simulink model "MATLAB_Arduino_ICM20689"  (R2021a)
settings: Solver=FixedStepAuto  StartTime=0.0  StopTime=300  RelTol=1e-3  EnableMultiTasking=on
undefined symbols (not defined in the file or in its folder): DiscIntNeverNeededParam
libraries: arduinolib x10
settings Model: SILPILModeSetting=veronly  ExtModeTrigDuration=2  Creator=mpnoy  LastModifiedBy=mpnoy
settings OptimizationCC: EnhancedBackFolding=on  PassReuseOutputArgsAs=Individual arguments  ZeroExternalMemoryAtStartup=off  ZeroInternalMemoryAtStartup=off  MaxStackSize=64  OptimizeBlockOrder=speed  DifferentSizesBufferReuse=on  OptimizationCustomize=off  EfficientTunableParamExpr=on
settings DebuggingCC: ParameterTunabilityLossMsg=error
settings HardwareCC: ProdBitPerInt=16  ProdBitPerPointer=16  ProdBitPerSizeT=16  ProdBitPerPtrDiffT=16  ProdLargestAtomicFloat=None  ProdWordSize=8  ProdHWDeviceType=Atmel->AVR
settings SFSimCC: MATLABDynamicMemAlloc=off
settings RTWCC: SystemTargetFile=ert.tlc  HardwareBoard=Arduino Uno  TemplateMakefile=ert_default_tmf  Toolchain=Arduino AVR  BuildConfiguration=Faster Runs
settings CodeAppCC: ForceParamTrailComments=on  IgnoreCustomStorageClasses=off  OperatorAnnotations=on  SimulinkDataObjDesc=on  SFDataObjDesc=on  InsertBlockDesc=on
settings ERTTargetCC: SupportContinuousTime=on  SupportVariableSizeSignals=on  ExtModeStaticAllocSize=250

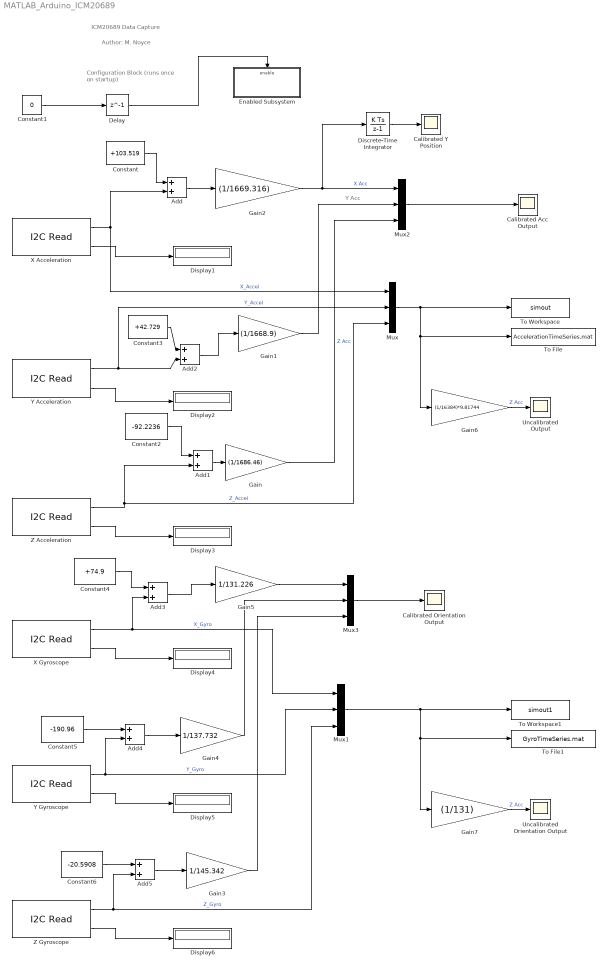
== system MATLAB_Arduino_ICM20689 ==
  note: Y Acc
  note: Author: M. Noyce
  note: ICM20689 Data Capture
  note: Configuration Block
      | (runs once on startup)
  Add{,1..5} (6 alike) : Sum
  "Calibrated Acc Output " : Scope
  Calibrated Orientation Output : Scope
  Calibrated Y Position : Scope
  Constant : Constant  Value=+103.519
  Constant1 : Constant  Value=0
  Constant2 : Constant  Value=-92.2236
  Constant3 : Constant  Value=+42.729
  Constant4 : Constant  Value=+74.9
  Constant5 : Constant  Value=-190.96
  Constant6 : Constant  Value=-20.5908
  Delay : Delay  DelayLength=1  InitialCondition=1
  Discrete-Time Integrator : DiscreteIntegrator  SampleTime=-1  ICPrevOutput=DiscIntNeverNeededParam  ICPrevScaledInput=DiscIntNeverNeededParam
  Display{1..6} (6 alike) : Display
  Enabled Subsystem : Subsystem  TreatAsAtomicUnit=on
  Gain : Gain  Gain=(1/1686.46)
  Gain1 : Gain  Gain=(1/1668.9)
  Gain2 : Gain  Gain=(1/1669.316)
  Gain3 : Gain  Gain=1/145.342
  Gain4 : Gain  Gain=1/137.732
  Gain5 : Gain  Gain=1/131.226
  Gain6 : Gain  Gain=(1/16384)*9.81744
  Gain7 : Gain  Gain=(1/131)
  Mux{,1..3} (4 alike) : Mux  Inputs=3
  To File : ToFile  Filename=AccelerationTimeSeries.mat  MatrixName=Acceleration  SaveFormat=Timeseries
  To File1 : ToFile  Filename=GyroTimeSeries.mat  MatrixName=Orientation  SaveFormat=Timeseries
  To Workspace : ToWorkspace  VariableName=simout  SaveFormat=Timeseries  SampleTime=-1
  To Workspace1 : ToWorkspace  VariableName=simout1  SaveFormat=Timeseries  SampleTime=-1
  "Uncalibrated Orientation Output " : Scope
  "Uncalibrated Output " : Scope
  "X Acceleration " : arduinolib/I2C Read  I2CModule=0  Mode=Master  SlaveAddress=104  SlaveByteOrder=BigEndian  Direction=Receiver  RegisterAddressMode=on  RegisterAddress=uint8(hex2dec('3B'))  SlaveDataType=int16  DataLength=1  NoAck=off  RepeatedStart=off  OutputStatus=on  blockPlatform=ARDUINO  SampleTime=0.01
      settings: SourceProductBaseCode=ARDUINO
  X Gyroscope : arduinolib/I2C Read  I2CModule=0  Mode=Master  SlaveAddress=104  SlaveByteOrder=BigEndian  Direction=Receiver  RegisterAddressMode=on  RegisterAddress=uint8(hex2dec('43'))  SlaveDataType=int16  DataLength=1  NoAck=off  RepeatedStart=off  OutputStatus=on  blockPlatform=ARDUINO  SampleTime=0.01
      settings: SourceProductBaseCode=ARDUINO
  Y Acceleration : arduinolib/I2C Read  I2CModule=0  Mode=Master  SlaveAddress=104  SlaveByteOrder=BigEndian  Direction=Receiver  RegisterAddressMode=on  RegisterAddress=uint8(hex2dec('3D'))  SlaveDataType=int16  DataLength=1  NoAck=off  RepeatedStart=off  OutputStatus=on  blockPlatform=ARDUINO  SampleTime=0.01
      settings: SourceProductBaseCode=ARDUINO
  Y Gyroscope : arduinolib/I2C Read  I2CModule=0  Mode=Master  SlaveAddress=104  SlaveByteOrder=BigEndian  Direction=Receiver  RegisterAddressMode=on  RegisterAddress=uint8(hex2dec('45'))  SlaveDataType=int16  DataLength=1  NoAck=off  RepeatedStart=off  OutputStatus=on  blockPlatform=ARDUINO  SampleTime=0.01
      settings: SourceProductBaseCode=ARDUINO
  "Z Acceleration " : arduinolib/I2C Read  I2CModule=0  Mode=Master  SlaveAddress=104  SlaveByteOrder=BigEndian  Direction=Receiver  RegisterAddressMode=on  RegisterAddress=uint8(hex2dec('3F'))  SlaveDataType=int16  DataLength=1  NoAck=off  RepeatedStart=off  OutputStatus=on  blockPlatform=ARDUINO  SampleTime=0.01
      settings: SourceProductBaseCode=ARDUINO
  Z Gyroscope : arduinolib/I2C Read  I2CModule=0  Mode=Master  SlaveAddress=104  SlaveByteOrder=BigEndian  Direction=Receiver  RegisterAddressMode=on  RegisterAddress=uint8(hex2dec('47'))  SlaveDataType=int16  DataLength=1  NoAck=off  RepeatedStart=off  OutputStatus=on  blockPlatform=ARDUINO  SampleTime=0.01
      settings: SourceProductBaseCode=ARDUINO
  wires:
  Constant1/1 -> Delay/1
  Delay/1 -> Enabled Subsystem/Enable
  "X Acceleration "/2 -> Display1/1
  Y Acceleration/2 -> Display2/1
  "Z Acceleration "/2 -> Display3/1
  "X Acceleration "/1 -> Add/2, Mux/1  "X_Accel"
  Y Acceleration/1 -> Mux/2, Add2/2  "Y_Accel"
  Mux/1 -> Gain6/1, To File/1, To Workspace/1
  "Z Acceleration "/1 -> Add1/2, Mux/3  "Z_Accel"
  Gain4/1 -> Mux3/2
  Gain3/1 -> Mux3/3
  Y Gyroscope/1 -> Add4/2, Mux1/2  "Y_Gyro"
  Z Gyroscope/1 -> Add5/2, Mux1/3  "Z_Gyro"
  X Gyroscope/1 -> Add3/2, Mux1/1  "X_Gyro"
  Gain5/1 -> Mux3/1
  Y Gyroscope/2 -> Display5/1
  Z Gyroscope/2 -> Display6/1
  X Gyroscope/2 -> Display4/1
  Constant/1 -> Add/1
  Constant2/1 -> Add1/1
  Gain/1 -> Mux2/3  "Z Acc"
  Add1/1 -> Gain/1
  Gain2/1 -> Discrete-Time Integrator/1, Mux2/1  "X Acc"
  Add/1 -> Gain2/1
  Constant3/1 -> Add2/1
  Add2/1 -> Gain1/1
  Gain1/1 -> Mux2/2
  Gain6/1 -> "Uncalibrated Output "/1  "Z Acc"
  Add3/1 -> Gain5/1
  Constant4/1 -> Add3/1
  Add4/1 -> Gain4/1
  Constant5/1 -> Add4/1
  Add5/1 -> Gain3/1
  Constant6/1 -> Add5/1
  Gain7/1 -> "Uncalibrated Orientation Output "/1  "Z Acc"
  Mux1/1 -> Gain7/1, To File1/1, To Workspace1/1
  Mux3/1 -> Calibrated Orientation Output/1
  Mux2/1 -> "Calibrated Acc Output "/1
  Discrete-Time Integrator/1 -> Calibrated Y Position/1

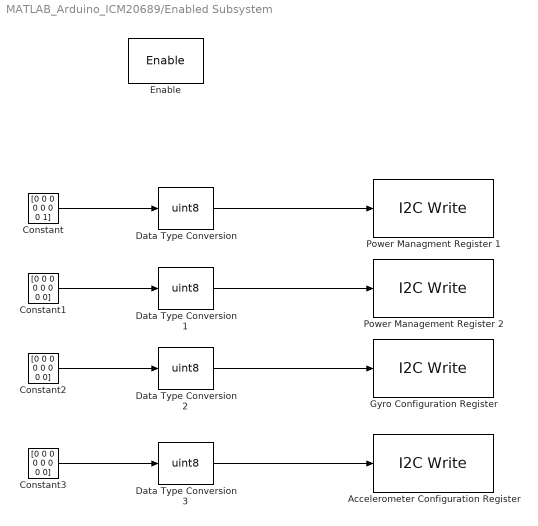
== system MATLAB_Arduino_ICM20689/Enabled Subsystem ==
  Enable : EnablePort
  "Accelerometer Configuration Register " : arduinolib/I2C Write  I2CModule=0  Mode=Master  SlaveAddress=104  SlaveByteOrder=BigEndian  Direction=Transmitter  RegisterAddressMode=on  RegisterAddress=uint8(hex2dec('1C'))  SlaveDataType=uint8  DataLength=1  NoAck=off  RepeatedStart=off  OutputStatus=off  blockPlatform=ARDUINO
      settings: SourceProductBaseCode=ARDUINO
  Constant : Constant  Value=[0 0 0 0 0 0 0 1]
  Constant1 : Constant  Value=[0 0 0 0 0 0 0 0]
  Constant2 : Constant  Value=[0 0 0 0 0 0 0 0]
  Constant3 : Constant  Value=[0 0 0 0 0 0 0 0]
  Data Type Conversion{,1..3} (4 alike) : DataTypeConversion  OutDataTypeStr=uint8
  Gyro Configuration Register : arduinolib/I2C Write  I2CModule=0  Mode=Master  SlaveAddress=104  SlaveByteOrder=BigEndian  Direction=Transmitter  RegisterAddressMode=on  RegisterAddress=uint8(hex2dec('1B'))  SlaveDataType=uint8  DataLength=1  NoAck=off  RepeatedStart=off  OutputStatus=off  blockPlatform=ARDUINO
      settings: SourceProductBaseCode=ARDUINO
  Power Management Register 2 : arduinolib/I2C Write  I2CModule=0  Mode=Master  SlaveAddress=104  SlaveByteOrder=BigEndian  Direction=Transmitter  RegisterAddressMode=on  RegisterAddress=uint8(hex2dec('6C'))  SlaveDataType=uint8  DataLength=1  NoAck=off  RepeatedStart=off  OutputStatus=off  blockPlatform=ARDUINO
      settings: SourceProductBaseCode=ARDUINO
  "Power Managment Register 1 " : arduinolib/I2C Write  I2CModule=0  Mode=Master  SlaveAddress=104  SlaveByteOrder=BigEndian  Direction=Transmitter  RegisterAddressMode=on  RegisterAddress=uint8(hex2dec('6B'))  SlaveDataType=uint8  DataLength=1  NoAck=off  RepeatedStart=off  OutputStatus=off  blockPlatform=ARDUINO
      settings: SourceProductBaseCode=ARDUINO
  wires:
  Data Type Conversion/1 -> "Power Managment Register 1 "/1
  Constant/1 -> Data Type Conversion/1
  Constant1/1 -> Data Type Conversion1/1
  Data Type Conversion1/1 -> Power Management Register 2/1
  Data Type Conversion2/1 -> Gyro Configuration Register/1
  Constant2/1 -> Data Type Conversion2/1
  Data Type Conversion3/1 -> "Accelerometer Configuration Register "/1
  Constant3/1 -> Data Type Conversion3/1
